simulink model "sl_robust_mobile_robot"  (R2024a)
settings: Solver=ode4  StartTime=0.0  StopTime=40.0  FixedStep=0.02  RelTol=1e-3
StopFcn:
  | if exist('yout','var'), q_s = yout(:,1:3); q_r = yout(:,4:8); err_s = hypot(q_r(:,1)-q_s(:,1), q_r(:,2)-q_s(:,2)); f_s = findobj('Type','figure','Name','Ket qua Chay Simulink (EKF + PID)'); if isempty(f_s), f_s = figure('Name','Ket qua Chay Simulink (EKF + PID)','NumberTitle','off','Color','w','Position',[180 100 940 420]); else, figure(f_s); clf(f_s); end; subplot(1,2,1); plot(q_r(:,1),q_r(:,2),'k:','LineWidth',2); hold on; grid on; plot(q_s(:,1),q_s(:,2),'g-','LineWidth',2); plot(q_s(1,1),q_s(1,2),'ro','MarkerFaceColor','r'); axis equal; xlim([-4.2 4.2]); ylim([-2.7 2.7]); xlabel('X [m]'); ylabel('Y [m]'); title('(a) Quy dao XY Robot chay tren Simulink (EKF + PID)'); legend('Tham chieu','Thuc te (EKF + PID)','Xuat phat','Location','southoutside'); subplot(1,2,2); plot(tout, err_s, 'b-', 'LineWidth', 1.6); grid on; xlim([0 40]); ylim([0 0.72]); xlabel('Thoi gian t [s]'); ylabel('Sai so ||e_p|| [m]'); title(sprintf('(b) Sai so bam vi tri (RMSE = %.4f m)', rms(err_s(tout>=3)))); end; open_system('sl_robust_mobile_robot/Pose_Scope');
libraries: slpidlib x2, simulink x1
settings Model: Creator=thuan  LastModifiedBy=thuan
settings DataIOCC: SaveFormat=Array

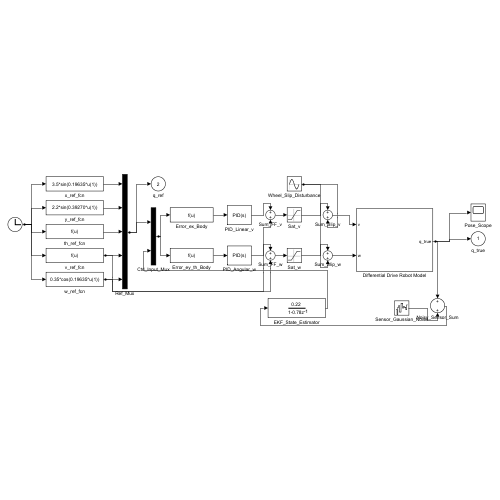
[thumbnail: Simulink's stored preview of the top-level diagram]
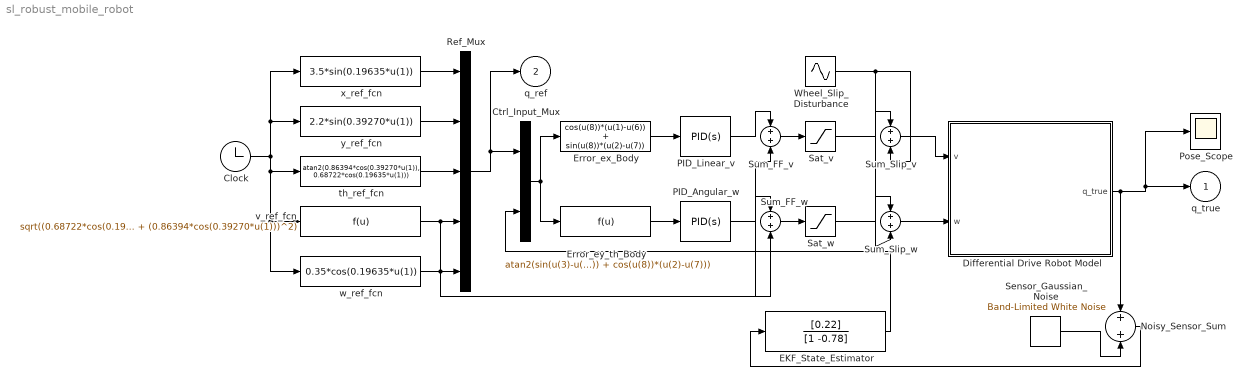
== system sl_robust_mobile_robot ==
  Clock : Clock
  Ctrl_Input_Mux : Mux  Inputs=2
  Differential Drive Robot Model : Subsystem
  EKF_State_Estimator : DiscreteFilter  Numerator=[0.22]  Denominator=[1 -0.78]  SampleTime=0.02
  Error_ex_Body : Fcn  Expr=cos(u(8))*(u(1)-u(6)) + sin(u(8))*(u(2)-u(7))
  Error_ey_th_Body : Fcn  Expr=atan2(sin(u(3)-u(8)),cos(u(3)-u(8))) + 1.25*u(4)*(-sin(u(8))*(u(1)-u(6)) + cos(u(8))*(u(2)-u(7)))
  Noisy_Sensor_Sum : Sum
  PID_Angular_w : slpidlib/PID Controller  Controller=PID  Form=Parallel  TimeDomain=Continuous-time  UseExternalTs=off  SampleTime=-1  IntegratorMethod=Forward Euler  FilterMethod=Forward Euler  ControllerParametersSource=internal  P=3.4  I=1.25  UseKiTs=off  D=0.15  UseExternalDerivativeSource=off  N=15  UseFilter=on  TunerSelectOption=Transfer Function Based (PID Tuner App)  InitialConditionSource=internal  InitialConditionForIntegrator=0  InitialConditionForFilter=0  DifferentiatorICPrevScaledInput=0  ExternalReset=none  TrackingMode=off  Kt=1  LimitOutput=off  SatLimitsSource=internal  UpperSaturationLimit=inf  LowerSaturationLimit=-inf  LinearizeAsGain=on  AntiWindupMode=none  Kb=1  LimitIntegrator=off  UpperIntegratorSaturationLimit=inf  LowerIntegratorSaturationLimit=-inf  POutMin=[]  POutMax=[]  IOutMin=[]  IOutMax=[]  DOutMin=[]  DOutMax=[]  NOutMin=[]  NOutMax=[]  SumOutMin=[]  SumOutMax=[]  SaturationOutMin=[]  SaturationOutMax=[]  PParamMin=[]  PParamMax=[]  IParamMin=[]  IParamMax=[]  DParamMin=[]  DParamMax=[]  NParamMin=[]  NParamMax=[]  KbParamMin=[]  KbParamMax=[]  KtParamMin=[]  KtParamMax=[]  KbOutMin=[]  KbOutMax=[]  KtOutMin=[]  KtOutMax=[]  IntegratorOutMin=[]  IntegratorOutMax=[]  FilterOutMin=[]  FilterOutMax=[]  SumI1OutMin=[]  SumI1OutMax=[]  SumI2OutMin=[]  SumI2OutMax=[]  SumI3OutMin=[]  SumI3OutMax=[]  SumI4OutMin=[]  SumI4OutMax=[]  SumDOutMin=[]  SumDOutMax=[]  DifferentiatorOutMin=[]  DifferentiatorOutMax=[]  FilterDiffOutCoefMin=[]  FilterDiffOutCoefMax=[]  ReciprocalOutMin=[]  ReciprocalOutMax=[]  SumDenOutMin=[]  SumDenOutMax=[]  SumNumOutMin=[]  SumNumOutMax=[]  DivideOutMin=[]  DivideOutMax=[]  UdiffTsProdOutMin=[]  UdiffTsProdOutMax=[]  NTsProdOutMin=[]  NTsProdOutMax=[]  UintegralTsProdOutMin=[]  UintegralTsProdOutMax=[]  UngainTsProdOutMin=[]  UngainTsProdOutMax=[]  ClampingZeroOutDataTypeStr=Inherit: Inherit via back propagation  ClampingZeroOutMin=[]  ClampingZeroOutMax=[]  FilterDenConstantOutDataTypeStr=Inherit: Inherit via back propagation  FilterDenConstantOutMin=[]  FilterDenConstantOutMax=[]  PCopyOutDataTypeStr=Inherit: Inherit via back propagation  PCopyOutMin=[]  PCopyOutMax=[]  NCopyOutDataTypeStr=Inherit: Inherit via back propagation  NCopyOutMin=[]  NCopyOutMax=[]  IntegratorContinuousStateAttributes=''  IntegratorStateMustResolveToSignalObject=off  IntegratorRTWStateStorageClass=Auto  FilterContinuousStateAttributes=''  FilterStateMustResolveToSignalObject=off  FilterRTWStateStorageClass=Auto  ParallelPVariant=InternalParameters  IdealPVariant=Disabled  IVariant=InternalParameters  DVariant=InternalParameters  IntegratorVariant=Continuous  SatVariant=Disabled  AWVariant=Passthrough  PCopyVariant=Disabled  TRVariant=Disabled  FdbkBlocksVariant=Forward  IdealPFdbkVariant=Disabled  SatFdbkVariant=Disabled  DerivativeFilterVariant=ContFilter  NVariant=InternalParameters  NCopyVariant=Disabled  FilterICVariant=InternalICsFilter  IntegratorICVariant=InternalICs  ExternalResetVariant=Disabled  TRSumVariant=Passthrough  SumFdbkVariant=Disabled  SumVariant=Sum_PID  TsampFilterVariant=InternalTs  TsampNgainVariant=Passthrough  TsampIntegralVariant=Disabled_SignalSpec  ExternalSaturationOutDataTypeStr=Inherit: Same as second input  DerivativeSourceVariant=ErrorSignal
  PID_Linear_v : slpidlib/PID Controller  Controller=PID  Form=Parallel  TimeDomain=Continuous-time  UseExternalTs=off  SampleTime=-1  IntegratorMethod=Forward Euler  FilterMethod=Forward Euler  ControllerParametersSource=internal  P=2.5  I=1.35  UseKiTs=off  D=0.12  UseExternalDerivativeSource=off  N=15  UseFilter=on  TunerSelectOption=Transfer Function Based (PID Tuner App)  InitialConditionSource=internal  InitialConditionForIntegrator=0  InitialConditionForFilter=0  DifferentiatorICPrevScaledInput=0  ExternalReset=none  TrackingMode=off  Kt=1  LimitOutput=off  SatLimitsSource=internal  UpperSaturationLimit=inf  LowerSaturationLimit=-inf  LinearizeAsGain=on  AntiWindupMode=none  Kb=1  LimitIntegrator=off  UpperIntegratorSaturationLimit=inf  LowerIntegratorSaturationLimit=-inf  POutMin=[]  POutMax=[]  IOutMin=[]  IOutMax=[]  DOutMin=[]  DOutMax=[]  NOutMin=[]  NOutMax=[]  SumOutMin=[]  SumOutMax=[]  SaturationOutMin=[]  SaturationOutMax=[]  PParamMin=[]  PParamMax=[]  IParamMin=[]  IParamMax=[]  DParamMin=[]  DParamMax=[]  NParamMin=[]  NParamMax=[]  KbParamMin=[]  KbParamMax=[]  KtParamMin=[]  KtParamMax=[]  KbOutMin=[]  KbOutMax=[]  KtOutMin=[]  KtOutMax=[]  IntegratorOutMin=[]  IntegratorOutMax=[]  FilterOutMin=[]  FilterOutMax=[]  SumI1OutMin=[]  SumI1OutMax=[]  SumI2OutMin=[]  SumI2OutMax=[]  SumI3OutMin=[]  SumI3OutMax=[]  SumI4OutMin=[]  SumI4OutMax=[]  SumDOutMin=[]  SumDOutMax=[]  DifferentiatorOutMin=[]  DifferentiatorOutMax=[]  FilterDiffOutCoefMin=[]  FilterDiffOutCoefMax=[]  ReciprocalOutMin=[]  ReciprocalOutMax=[]  SumDenOutMin=[]  SumDenOutMax=[]  SumNumOutMin=[]  SumNumOutMax=[]  DivideOutMin=[]  DivideOutMax=[]  UdiffTsProdOutMin=[]  UdiffTsProdOutMax=[]  NTsProdOutMin=[]  NTsProdOutMax=[]  UintegralTsProdOutMin=[]  UintegralTsProdOutMax=[]  UngainTsProdOutMin=[]  UngainTsProdOutMax=[]  ClampingZeroOutDataTypeStr=Inherit: Inherit via back propagation  ClampingZeroOutMin=[]  ClampingZeroOutMax=[]  FilterDenConstantOutDataTypeStr=Inherit: Inherit via back propagation  FilterDenConstantOutMin=[]  FilterDenConstantOutMax=[]  PCopyOutDataTypeStr=Inherit: Inherit via back propagation  PCopyOutMin=[]  PCopyOutMax=[]  NCopyOutDataTypeStr=Inherit: Inherit via back propagation  NCopyOutMin=[]  NCopyOutMax=[]  IntegratorContinuousStateAttributes=''  IntegratorStateMustResolveToSignalObject=off  IntegratorRTWStateStorageClass=Auto  FilterContinuousStateAttributes=''  FilterStateMustResolveToSignalObject=off  FilterRTWStateStorageClass=Auto  ParallelPVariant=InternalParameters  IdealPVariant=Disabled  IVariant=InternalParameters  DVariant=InternalParameters  IntegratorVariant=Continuous  SatVariant=Disabled  AWVariant=Passthrough  PCopyVariant=Disabled  TRVariant=Disabled  FdbkBlocksVariant=Forward  IdealPFdbkVariant=Disabled  SatFdbkVariant=Disabled  DerivativeFilterVariant=ContFilter  NVariant=InternalParameters  NCopyVariant=Disabled  FilterICVariant=InternalICsFilter  IntegratorICVariant=InternalICs  ExternalResetVariant=Disabled  TRSumVariant=Passthrough  SumFdbkVariant=Disabled  SumVariant=Sum_PID  TsampFilterVariant=InternalTs  TsampNgainVariant=Passthrough  TsampIntegralVariant=Disabled_SignalSpec  ExternalSaturationOutDataTypeStr=Inherit: Same as second input  DerivativeSourceVariant=ErrorSignal
  Pose_Scope : Scope
  Ref_Mux : Mux  Inputs=5
  Sat_v : Saturate  UpperLimit=1.8  LowerLimit=-1.8
  Sat_w : Saturate  UpperLimit=3.0  LowerLimit=-3.0
  Sensor_Gaussian_Noise : simulink/Sources/Band-Limited White Noise  Cov=[0.0004 0.0004 0.0001]  Ts=0.02  seed=[11 22 33]
  Sum_FF_v : Sum
  Sum_FF_w : Sum
  Sum_Slip_v : Sum
  Sum_Slip_w : Sum
  Wheel_Slip_Disturbance : Sin  Amplitude=0.14  Bias=-0.06  Frequency=1.4  SampleTime=0
  th_ref_fcn : Fcn  Expr=atan2(0.86394*cos(0.39270*u(1)), 0.68722*cos(0.19635*u(1)))
  v_ref_fcn : Fcn  Expr=sqrt((0.68722*cos(0.19635*u(1)))^2 + (0.86394*cos(0.39270*u(1)))^2)
  w_ref_fcn : Fcn  Expr=0.35*cos(0.19635*u(1))
  x_ref_fcn : Fcn  Expr=3.5*sin(0.19635*u(1))
  y_ref_fcn : Fcn  Expr=2.2*sin(0.39270*u(1))
  q_true : Outport
  q_ref : Outport  Port=2
  wires:
  Clock/1 -> v_ref_fcn/1, w_ref_fcn/1, th_ref_fcn/1, x_ref_fcn/1, y_ref_fcn/1
  x_ref_fcn/1 -> Ref_Mux/1
  y_ref_fcn/1 -> Ref_Mux/2
  th_ref_fcn/1 -> Ref_Mux/3
  v_ref_fcn/1 -> Ref_Mux/4, Sum_FF_v/2
  w_ref_fcn/1 -> Ref_Mux/5, Sum_FF_w/2
  Ref_Mux/1 -> Ctrl_Input_Mux/1, q_ref/1
  Ctrl_Input_Mux/1 -> Error_ex_Body/1, Error_ey_th_Body/1
  Error_ex_Body/1 -> PID_Linear_v/1
  Error_ey_th_Body/1 -> PID_Angular_w/1
  PID_Linear_v/1 -> Sum_FF_v/1
  PID_Angular_w/1 -> Sum_FF_w/1
  Sum_FF_v/1 -> Sat_v/1
  Sum_FF_w/1 -> Sat_w/1
  Sat_v/1 -> Sum_Slip_v/1
  Wheel_Slip_Disturbance/1 -> Sum_Slip_v/2, Sum_Slip_w/2
  Sat_w/1 -> Sum_Slip_w/1
  Sum_Slip_v/1 -> Differential Drive Robot Model/1(v)
  Sum_Slip_w/1 -> Differential Drive Robot Model/2(w)
  Differential Drive Robot Model/1(q_true) -> q_true/1, Pose_Scope/1, Noisy_Sensor_Sum/1
  Sensor_Gaussian_Noise/1 -> Noisy_Sensor_Sum/2
  Noisy_Sensor_Sum/1 -> EKF_State_Estimator/1
  EKF_State_Estimator/1 -> Ctrl_Input_Mux/2

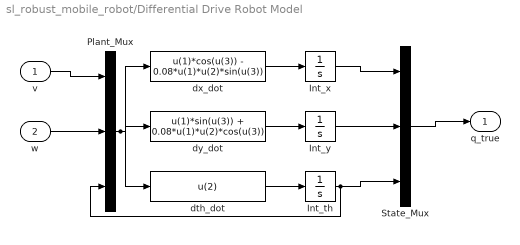
== system sl_robust_mobile_robot/Differential Drive Robot Model ==
  v : Inport
  w : Inport  Port=2
  Int_th : Integrator  InitialCondition=0.50
  Int_x : Integrator  InitialCondition=0.40
  Int_y : Integrator  InitialCondition=-0.45
  Plant_Mux : Mux  Inputs=3
  State_Mux : Mux  Inputs=3
  dth_dot : Fcn  Expr=u(2)
  dx_dot : Fcn  Expr=u(1)*cos(u(3)) - 0.08*u(1)*u(2)*sin(u(3))
  dy_dot : Fcn  Expr=u(1)*sin(u(3)) + 0.08*u(1)*u(2)*cos(u(3))
  q_true : Outport
  wires:
  v/1 -> Plant_Mux/1
  w/1 -> Plant_Mux/2
  Int_th/1 -> Plant_Mux/3, State_Mux/3
  Plant_Mux/1 -> dx_dot/1, dy_dot/1, dth_dot/1
  dx_dot/1 -> Int_x/1
  dy_dot/1 -> Int_y/1
  dth_dot/1 -> Int_th/1
  Int_x/1 -> State_Mux/1
  Int_y/1 -> State_Mux/2
  State_Mux/1 -> q_true/1
